simulink model "solar_car"  (R2025b)
settings: Solver=VariableStepAuto  StartTime=0.0  StopTime=10.0  RelTol=1e-3
undefined symbols (not defined in the file or in its folder): Ion, Lithium
libraries: spsBatteryLib x3, spsControlledVoltageSourceLib x2, spsPVArrayLib x2, BatteryEstimators x1, spsCurrentMeasurementLib x1, BatteryBalancing x1, simulink x1, spsVoltageMeasurementLib x1, spspowerguiLib x1
settings Model: Creator=jonat  LastModifiedBy=jonat

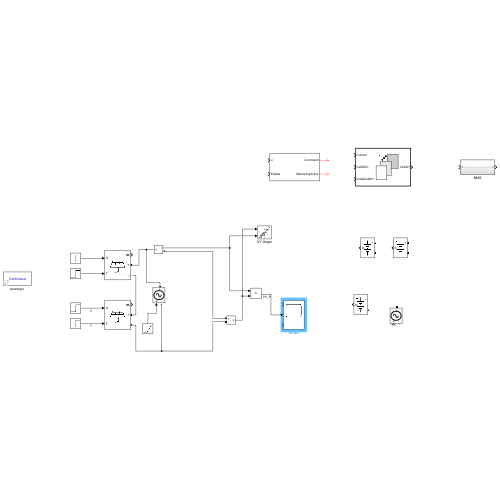
[thumbnail: Simulink's stored preview of the top-level diagram]
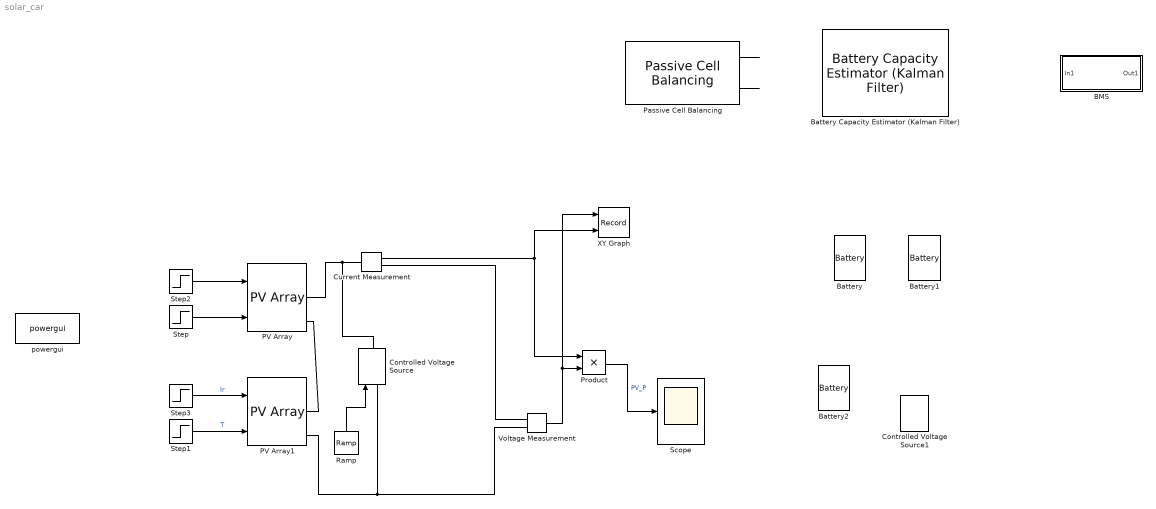
== system solar_car ==
  BMS : Subsystem
  Battery : spsBatteryLib/Battery  BatType=Lithium-Ion  NomV=7.2  NomQ=5.4  SOC=100  Batt_Tr=30  PresetModel=on  MaxQ=5.4  MinV=5.4  FullV=8.3807  Dis_rate=2.3478  R=0.013333  Normal_OP=4.8835  expZone="[7.7788      0.2653]"
  Battery Capacity Estimator (Kalman Filter) : BatteryEstimators/Battery Capacity Estimator (Kalman Filter)  CurrentInputPartition=off  filterType=Extended Kalman filter  alpha=1  beta=2  kappa=0  Q=3e-4  R=5e-7  P0=1e-8  Ts=1  DataType=Inherit: auto
      settings: LibrarySourceBlock=|
      | batt_sl_lib/Estimators/Battery Capacity Estimator
      | (Kalman Filter)
  Battery1 : spsBatteryLib/Battery  BatType=Lithium-Ion  NomV=7.2  NomQ=5.4  SOC=100  Batt_Tr=30  PresetModel=on  MaxQ=5.4  MinV=5.4  FullV=8.3807  Dis_rate=2.3478  R=0.013333  Normal_OP=4.8835  expZone="[7.7788      0.2653]"
  Battery2 : spsBatteryLib/Battery  BatType=Lithium-Ion  NomV=7.2  NomQ=5.4  SOC=100  Batt_Tr=30  PresetModel=on  MaxQ=5.4  MinV=5.4  FullV=8.3807  Dis_rate=2.3478  R=0.013333  Normal_OP=4.8835  expZone="[7.7788      0.2653]"
  Controlled Voltage Source : spsControlledVoltageSourceLib/Controlled Voltage Source  Initialize=on  Source_Type=AC  Amplitude=0  Phase=0  Frequency=0  Measurements=None
  Controlled Voltage Source1 : spsControlledVoltageSourceLib/Controlled Voltage Source  Initialize=on  Source_Type=AC  Amplitude=0  Phase=0  Frequency=0  Measurements=None
  Current Measurement : spsCurrentMeasurementLib/Current Measurement  PhasorSimulation=off  OutputType=Complex  PSBequivalent=0
  PV Array : spsPVArrayLib/PV Array  Npar=1  Nser=1  PlotType=array @ 25 deg.C & specified irradiances  S_vec="[ 1000  500  100 ]"  Temp_C_vec="[ 45 25  ]"  ModuleName=User-defined  PlotWhenSelected=off  Pm=4.14  Ncell=18  Voc=10.9  Isc=0.495  Vm=9  Im=0.46  beta_Voc_pc=-0.37  alpha_Isc_pc=0.102  beta_Voc=-0.04033  alpha_Isc=0.0005049  IL=0.49567  I0=2.498e-11  nI=0.99514  Rsh=848.6941  Rs=1.1458  RobustModel=off  RobustCellTemperature=313.3991  BAL=on  Tc=1e-6  Tfilter=5e-5
  PV Array1 : spsPVArrayLib/PV Array  Npar=1  Nser=1  PlotType=array @ 25 deg.C & specified irradiances  S_vec="[ 1000  500  100 ]"  Temp_C_vec="[ 45 25  ]"  ModuleName=User-defined  PlotWhenSelected=off  Pm=4.14  Ncell=18  Voc=10.9  Isc=0.495  Vm=9  Im=0.46  beta_Voc_pc=-0.37  alpha_Isc_pc=0.102  beta_Voc=-0.04033  alpha_Isc=0.0005049  IL=0.49567  I0=2.498e-11  nI=0.99514  Rsh=848.6941  Rs=1.1458  RobustModel=off  RobustCellTemperature=313.3991  BAL=on  Tc=1e-6  Tfilter=5e-5
  Passive Cell Balancing : BatteryBalancing/Passive Cell Balancing  Threshold=0.2  HysteresisBand=0  Td_on=1  Td_off=1  Ts=1  dataType=double
      settings: LibrarySourceBlock=batt_sl_lib/Cell Balancing/Passive Cell Balancing
  Product : Product
  Ramp : simulink/Sources/Ramp  slope=21.8  start=0  InitialOutput=0
  Scope : Scope  NumInputPorts=3
      settings: ActiveDisplayYMinimum=-1.4612380091265695E-14  ActiveDisplayYMaximum=1.3151142082139129E-13
  Step : Step  Time=0  After=25  SampleTime=0
  Step1 : Step  Time=0  After=25  SampleTime=0
  Step2 : Step  Time=0  After=1000  SampleTime=0
  Step3 : Step  Time=0  After=1000  SampleTime=0
  Voltage Measurement : spsVoltageMeasurementLib/Voltage Measurement  PhasorSimulation=off  OutputType=Complex  PSBequivalent=0
  XY Graph : Record  NumPorts=2.0  FileSettingsInternal="{\"entries\":[{\"content\":{\"excelSettings\":{\"content\":{},\"type\":\"Streamout.ExcelSettings\"},\"parquetSettings\":{\"content\":{},\"type\":\"Streamout.ParquetSettings\"}},\"type\":\"Streamout.FileSettingStorage\",\"uuid\":\"\"}],\"packageUris\":[\"http:\\/\\/schema.mathworks.com\\/mf0\\/streamout_blocks\\/R2020a\"],\"version\":\"1.0\"}"  FrameSettings=[0, 0]  Layout=[1 1]  SignalsInternal="{\"entries\":[{\"content\":{\"signals\":[{\"content\":{\"blockPath\":[],\"dimensions\":[1],\"domain\":\"\",\"lineColor\":\"#a2142f\",\"plots\":[ 1 ],\"port\":1,\"signalID\":1,\"signalName\":\"Voltage Measurement\"},\"type\":\"RecordBlkView.Signal\",\"uuid\":\"\"},{\"content\":{\"blockPath\":[],\"dimensions\":[1],\"domain\":\"\",\"lineColor\":\"#139fff\",\"plots\":[ 1 ],\"port\":2,\"signalID\":2,\"signalName\":\"Current Measurement\"},\"type\":\"RecordBlkView.Signal\",\"uuid\":\"\"}]},\"type\":\"RecordBlkView.InputSignals\",\"uuid\":\"\"}],\"packageUris\":[\"http:\\/\\/schema.mathworks.com\\/mf0\\/streamout_blocks\\/R2020a\"],\"version\":\"1.0\"}"  VisualizationBindings="{\"xyplotplugin\":{\"info\":[{\"series\":[{\"bindingParametersList\":[{\"parameter\":\"X-Axis\",\"signalID\":1,\"signalName\":\"Voltage Measurement\"},{\"parameter\":\"Y-Axis\",\"signalID\":2,\"signalName\":\"Current Measurement\"}],\"seriesID\":0}],\"subplotID\":1}]}}"  CompatibilityTag=XY
  powergui : spspowerguiLib/powergui  Priority=1  SimulationMode=Continuous  SampleTime=50e-6  frequency=60  Iterations=50  frequencyindice=0  Pbase=100e6  ErrMax=1e-4  UnitsV=kV  UnitsW=MW  buscounter=0  FunctionMessages=off  echomessages=off  EnableUseOfTLC=off  CurrentSourceSwitches=off  DisableSnubberDevices=off  DisableRonSwitches=off  DisableVfSwitches=off  DisplayEquations=off  AutomaticDiscreteSolvers=off  SolverType=Tustin/Backward Euler (TBE)  Interpol=off  ExternalGateDelay=off  methode=off  Ts=100  x0status=blocks  SPID=on  SwTol=0  HookPort=off  NonlinearTolerance=1e-4  nMaxIteration=100  ContinueOnMaxIteration=off  RestoreLinks=warning  ResistiveCurrentMeasurement=off  Frange=[0:2:500]  Ylog=off  Xlog=on  ShowGrid=off  save=off  variable=ZData  structure=0  ZoomFFT=off  StartTime=0.0  cycles=1  DisplayStyle=1  fundamental=60  FreqAxis=off  MaxFrequency=1000  frequencyindicesteady=1  RmsSteady=1  display=off
  wires:
  Passive Cell Balancing/1 -> ?
  Passive Cell Balancing/2 -> ?
  Step/1 -> PV Array/2
  Step2/1 -> PV Array/1
  Step3/1 -> PV Array1/1  "Ir"
  Step1/1 -> PV Array1/2  "T"
  Ramp/1 -> Controlled Voltage Source/1
  Current Measurement/1 -> Product/1, XY Graph/2
  Voltage Measurement/1 -> XY Graph/1, Product/2
  Product/1 -> Scope/2  "PV_P"
  connections:
  Voltage Measurement/LConn2 -- Controlled Voltage Source/LConn1 -- PV Array1/RConn2
  PV Array/RConn1 -- Controlled Voltage Source/RConn1 -- Current Measurement/LConn1
  PV Array1/RConn1 -- PV Array/RConn2
  Current Measurement/RConn1 -- Voltage Measurement/LConn1

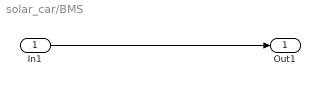
== system solar_car/BMS ==
  In1 : Inport
  Out1 : Outport
  wires:
  In1/1 -> Out1/1
